simulink model "Lab04_Group06_model"  (R2022b)
settings: Solver=ode1  StartTime=0.0  StopTime=10  FixedStep=0.002  RelTol=1e-3  EnableMultiTasking=on
undefined symbols (not defined in the file): DiscIntNeverNeededParam, HIL
libraries: quarc_library x6
settings Model: ExtModeTrigDuration=10000  Creator=hamzah.nadeem  LastModifiedBy=hamzah.nadeem
settings SolverCC: AlgebraicLoopSolver=TrustRegion  PositivePriorityOrder=on
settings DataIOCC: ReturnWorkspaceOutputs=off
settings DebuggingCC: UnconnectedInputMsg=warning  UnconnectedOutputMsg=warning  UnconnectedLineMsg=warning  SFMachineParentedDataDiag=warning  ArithmeticOperatorsInVariantConditions=warning
settings ModelReferenceCC: EnableRefExpFcnMdlSchedulingChecks=on
settings SFSimCC: SimUseLocalCustomCode=off  CustomCodeUndefinedFunction=UseInterfaceOnly
settings RTWCC: Description=QUARC Win64 Target Using Toolchain  SystemTargetFile=quarc_win64.tlc  TemplateMakefile=quarc_default_tmf  RTWUseLocalCustomCode=off  Toolchain=QUARC win64 | nmake (64-bit Windows)  BuildConfiguration=Faster Runs
settings CodeAppCC: StateflowObjectComments=on
settings STFCustomTargetCC: TargetLangStandard=C99 (ISO)  ConcurrentExecutionCompliant=on  GRTInterface=on  UseToolchainInfoCompliant=on  SystemTargetFile=quarc_win64.tlc
settings GRTTargetCC: ParMdlRefBuildCompliant=off  CompOptLevelCompliant=off  CombineOutputUpdateFcns=off  MatFileLogging=off  CPPClassGenCompliant=off  GRTInterface=on  ExtMode=on  ExtModeMexFile=quarc_comm
settings ConfigComp: CovMetricSettings=dswe

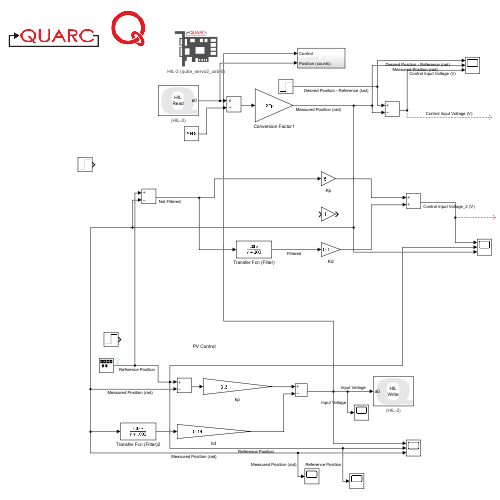
[thumbnail: Simulink's stored preview of the top-level diagram]
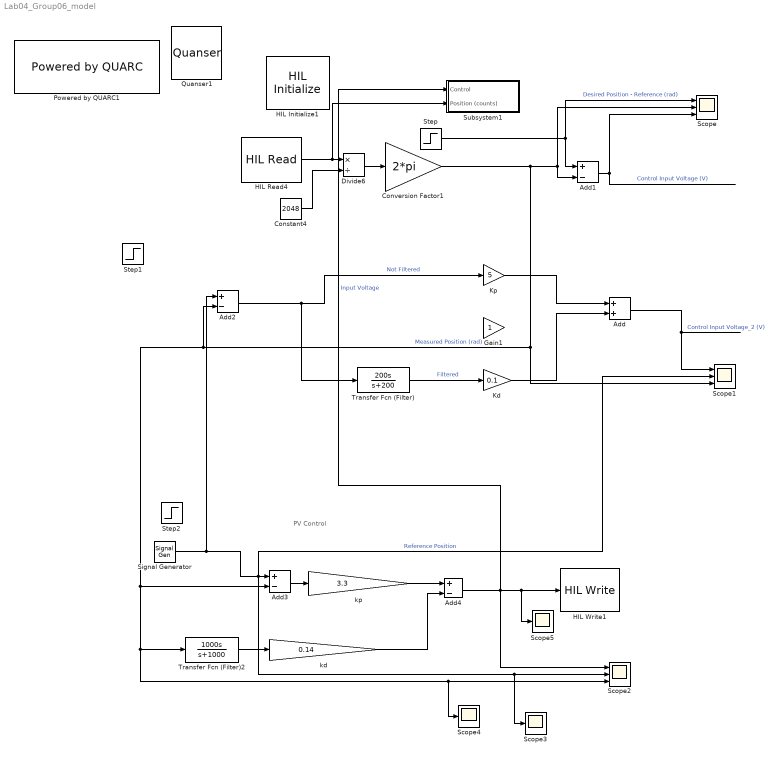
== system Lab04_Group06_model ==
  note: PV Control
  Add : Sum
  Add{1..4} (4 alike) : Sum  Inputs=+-
  Constant4 : Constant  Value=2048
  Conversion Factor1 : Gain  Gain=2*pi
  Divide6 : Product  Inputs=*/  RndMeth=Zero  SaturateOnIntegerOverflow=on
  Gain1 : Gain
  HIL Initialize1 : quarc_library/Data Acquisition/Generic/Configuration/HIL Initialize  object_name=HIL-2  board_type=qube_servo2_usb  board_number=0  board_options=""  exclusive=off  active=on  hardware_clocks=[0]  clock_modes=[]  initial_clock_frequencies=[]  set_clock_params_at_start=off  set_clock_params_at_switch_in=off  set_clock_frequencies_at_start=off  set_clock_frequencies_at_switch_in=off  analog_input_channels=[0]  analog_input_configurations=[]  analog_input_maximums=3  analog_input_minimums=-3  set_analog_input_params_at_start=off  set_analog_input_params_at_switch_in=off  analog_output_channels=[0]  analog_output_maximums=15  analog_output_minimums=-15  initial_analog_outputs=[0]  final_analog_outputs=[0]  watchdog_analog_outputs=0  set_analog_output_params_at_start=off  set_analog_output_params_at_switch_in=off  set_analog_outputs_at_start=on  set_analog_outputs_at_switch_in=off  set_analog_outputs_at_terminate=on  set_analog_outputs_at_switch_out=off  set_analog_outputs_on_watchdog=on  digital_input_channels=[]  digital_output_channels=[0]  digital_output_configuration=[]  initial_digital_outputs=[1]  final_digital_outputs=[0]  watchdog_digital_outputs=[0]  set_digital_output_params_at_start=off  set_digital_output_params_at_switch_in=off  set_digital_outputs_at_start=on  set_digital_outputs_at_switch_in=off  set_digital_outputs_at_terminate=on  set_digital_outputs_at_switch_out=off  set_digital_outputs_on_watchdog=on  encoder_channels=[0:1]  quadrature=[4]  encoder_filter_frequency=[]  initial_encoder_counts=[0]  set_encoder_params_at_start=off  set_encoder_params_at_switch_in=off  set_encoder_counts_at_start=on  set_encoder_counts_at_switch_in=off  pwm_channels=[]  pwm_modes=[]  pwm_frequency=[]  pwm_configuration=[]  pwm_alignment=[]  pwm_polarity=[]  pwm_leading_deadband=[]  pwm_trailing_deadband=[]  initial_pwm_outputs=[]  final_pwm_outputs=[]  watchdog_pwm_outputs=[]  set_pwm_params_at_start=off  set_pwm_params_at_switch_in=off  set_pwm_outputs_at_start=off  set_pwm_outputs_at_switch_in=off  set_pwm_outputs_at_terminate=off  set_pwm_outputs_at_switch_out=off  set_pwm_outputs_on_watchdog=off  other_output_channels=[11000:11002]  initial_other_outputs=[0 1 0]  final_other_outputs=[1 0 0]  watchdog_other_outputs=[0 0 1]  set_other_outputs_at_start=on  set_other_outputs_at_switch_in=off  set_other_outputs_at_terminate=on  set_other_outputs_at_switch_out=off  set_other_outputs_on_watchdog=on
  HIL Read4 : quarc_library/Data Acquisition/Generic/Immediate I//O/HIL Read  object_name=HIL-2  analog_channels=[]  encoder_channels=0  digital_channels=[]  other_channels=[]  sample_time=qc_get_step_size  active=on  vector_output=off  data_type_mode=Inherit via back propagation  encoder_data_type=double  digital_data_type=boolean
  HIL Write1 : quarc_library/Data Acquisition/Generic/Immediate I//O/HIL Write  object_name=HIL-2  analog_channels=0  pwm_channels=[]  digital_channels=[]  other_channels=[]  sample_time=-1  active=off  vector_input=off
  Kd : Gain  Gain=0.1
  Kp : Gain  Gain=5
  Powered by QUARC1 : quarc_library/Logos/Powered by QUARC
  Quanser1 : quarc_library/Logos/Quanser
  Scope : Scope  NumInputPorts=3
  Scope1 : Scope  NumInputPorts=3
  Scope2 : Scope  NumInputPorts=3
  Scope3 : Scope
  Scope4 : Scope
  Scope5 : Scope
  Signal Generator : SignalGenerator  WaveForm=square  Amplitude=0.5  Frequency=0.4
  Step : Step  SampleTime=0
  Step1 : Step  SampleTime=0
  Step2 : Step  SampleTime=0
  Subsystem1 : Subsystem
  Transfer Fcn (Filter) : TransferFcn  Numerator=[200 0]  Denominator=[1 200]
  Transfer Fcn (Filter)2 : TransferFcn  Numerator=[1000, 0]  Denominator=[1 1000]
  kd : Gain  Gain=0.14
  kp : Gain  Gain=3.3
  wires:
  Constant4/1 -> Divide6/2
  Divide6/1 -> Conversion Factor1/1
  HIL Read4/1 -> Subsystem1/2(Position (counts)), Divide6/1
  Add1/1 -> Scope/3  "Control Input Voltage (V)"
  Conversion Factor1/1 -> Scope1/3, Scope4/1, Scope2/3, Transfer Fcn (Filter)2/1, Add3/2, Add2/2, Add1/2, Scope/2  "Measured Position (rad)"
  Step/1 -> Add1/1, Scope/1  "Desired Position - Reference (rad)"
  Transfer Fcn (Filter)/1 -> Kd/1  "Filtered"
  Kp/1 -> Add/1
  Kd/1 -> Add/2
  Add2/1 -> Kp/1, Transfer Fcn (Filter)/1  "Not Filtered"
  Add/1 -> Scope1/1  "Control Input Voltage_2 (V)"
  Add3/1 -> kp/1
  kp/1 -> Add4/1
  Add4/1 -> Scope5/1, HIL Write1/1, Subsystem1/1(Control), Scope2/1  "Input Voltage"
  Signal Generator/1 -> Add2/1, Add3/1, Scope3/1, Scope2/2, Scope1/2  "Reference Position"
  Transfer Fcn (Filter)2/1 -> kd/1
  kd/1 -> Add4/2

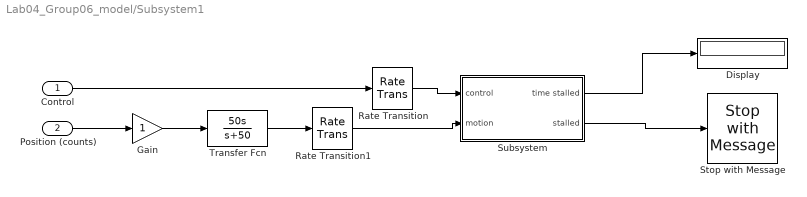
== system Lab04_Group06_model/Subsystem1 ==
  Control : Inport
  Position (counts) : Inport  Port=2
  Display : Display
  Gain : Gain
  Rate Transition : RateTransition
  Rate Transition1 : RateTransition
  Stop with Message : quarc_library/Sinks/Error Handling/Stop with Message  message_type=Fixed error message  message_icon=Error  message=Stall Detected! Please snsure that the DC motor is free to move and is functioning properly. Please ask a TA to check your code if you have recived this error.
  Subsystem : Subsystem
  Transfer Fcn : TransferFcn  Numerator=[50 0]  Denominator=[1 50]
  wires:
  Subsystem/2(stalled) -> Stop with Message/1
  Subsystem/1(time stalled) -> Display/1
  Rate Transition/1 -> Subsystem/1(control)
  Rate Transition1/1 -> Subsystem/2(motion)
  Transfer Fcn/1 -> Rate Transition1/1
  Gain/1 -> Transfer Fcn/1
  Position (counts)/1 -> Gain/1
  Control/1 -> Rate Transition/1

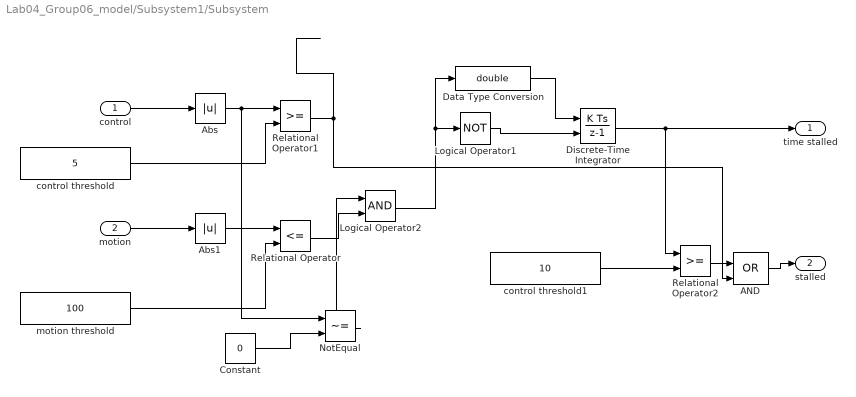
== system Lab04_Group06_model/Subsystem1/Subsystem ==
  control : Inport
  motion : Inport  Port=2
  AND : Logic  Operator=OR  IconShape=distinctive  AllPortsSameDT=off  OutDataTypeStr=boolean
  Abs : Abs  SaturateOnIntegerOverflow=off
  Abs1 : Abs  SaturateOnIntegerOverflow=off
  Constant : Constant  Value=0
  Data Type Conversion : DataTypeConversion  OutDataTypeStr=double  SaturateOnIntegerOverflow=off  RndMeth=Floor
  Discrete-Time Integrator : DiscreteIntegrator  ExternalReset=rising  SampleTime=-1  ICPrevOutput=DiscIntNeverNeededParam  ICPrevScaledInput=DiscIntNeverNeededParam
  Logical Operator1 : Logic  Operator=NOT  AllPortsSameDT=off  OutDataTypeStr=boolean
  Logical Operator2 : Logic  AllPortsSameDT=off  OutDataTypeStr=boolean
  NotEqual : RelationalOperator  Operator=~=  OutDataTypeStr=boolean  RndMeth=Simplest  InputSameDT=off
  Relational Operator : RelationalOperator  Operator=<=  OutDataTypeStr=boolean  InputSameDT=off
  Relational Operator1 : RelationalOperator  OutDataTypeStr=boolean  InputSameDT=off
  Relational Operator2 : RelationalOperator  OutDataTypeStr=boolean  InputSameDT=off
  control threshold : Constant  Value=5
  control threshold1 : Constant  Value=10
  motion threshold : Constant  Value=100
  time stalled : Outport
  stalled : Outport  Port=2
  wires:
  NotEqual/1 -> Logical Operator2/1
  Relational Operator/1 -> Logical Operator2/2
  AND/1 -> stalled/1
  Relational Operator2/1 -> AND/1
  Relational Operator1/1 -> AND/2
  Constant/1 -> NotEqual/2
  control threshold1/1 -> Relational Operator2/2
  Abs1/1 -> Relational Operator/1
  Data Type Conversion/1 -> Discrete-Time Integrator/1
  Discrete-Time Integrator/1 -> Relational Operator2/1, time stalled/1
  Logical Operator1/1 -> Discrete-Time Integrator/2
  control/1 -> Abs/1
  Abs/1 -> Relational Operator1/1, NotEqual/1
  control threshold/1 -> Relational Operator1/2
  motion threshold/1 -> Relational Operator/2
  Logical Operator2/1 -> Data Type Conversion/1, Logical Operator1/1
  motion/1 -> Abs1/1
